simulink model "PMSM_FOC_R2026a"  (R2026a)
settings: Solver=ode4  StopTime=0.25  FixedStep=timing_h  MaxStep=1e-6
InitFcn:
  | pmsm_sensorless_v2_init(bdroot);
model workspace (MATLAB code in the model file + MAT data in the model file):
  T = 1e-6    (= 1e-06)
  MotorProfile = 'CHENSHA 200W / firmware profile revision 2'
  MotorSourceCommit = '48d6e86814ac6657b1313b4c92ef24c88f492e07'
  Pn = 200
  Un = 24
  Vdc = 24
  I_rated_rms = 11.5
  I_peak_rms = 23
  In = sqrt(2)*I_rated_rms
  I_peak = sqrt(2)*I_peak_rms
  n = 3000
  p = 5
  Rs = 0.105125
  Ld = 103.7615e-6    (= 0.0001037615)
  Lq = 103.7615e-6    (= 0.0001037615)
  Ls = Ld    (= 0.0001037615)
  phis = 0.06/(sqrt(2)*1.5*p)
  J = 32e-6    (= 3.2e-05)
  F = 0
  Kt = 1.5*p*phis
  Tn = 0.69
  T_peak = 1.38
  Iq_limit = 8
  accel_limit_rad_s2 = 1200
  speed_peak_rad_s = 335
  I_protection_A = 10
  Vbus_protection_high_V = 30
  Vbus_protection_low_V = 10
  RE = 10000
  rr = 2*pi/RE    (= 0.000628318530718)
  encoder_direction = -1
  fN = p*n/60    (= 250)
  wN = 2*pi*fN    (= 1570.79632679)
  ki_p = 0.8
  ki_i = 1
  fc = 20e3    (= 20000)
  Ts = 1/fc    (= 5e-05)
  dt = Ts    (= 5e-05)
  Ts_speed = 2*dt    (= 0.0001)
  w_sb = 2*pi*fN*1.2    (= 1884.95559215)
  fcb = 1000
  fwb = 50
  wc = 2*pi*fcb    (= 6283.18530718)
  wsc = 2*pi*fwb    (= 314.159265359)
  K = 30/pi    (= 9.54929658551)
  kp_w = 0.00069087230807625508    (= 0.000690872308076)
  ki_w = 0.04340878735241975    (= 0.0434087873524)
  ks_w = 0.98718608264211138    (= 0.987186082642)
  kp_id = 0.7539822368615503    (= 0.753982236862)
  ki_id = 879.64594300514204    (= 879.645943005)
  ks_id = 1.1309733552923253    (= 1.13097335529)
  kp_iq = 0.7539822368615503    (= 0.753982236862)
  ki_iq = 879.64594300514204    (= 879.645943005)
  ks_iq = 1.1309733552923253    (= 1.13097335529)
  Bm = 0
  uplimit_w = Kt*Iq_limit
  downlimit_w = -uplimit_w
  uplimit_id = Vdc/sqrt(3)
  downlimit_id = -uplimit_id
  uplimit_iq = Vdc/sqrt(3)
  downlimit_iq = -uplimit_iq
  teaching_Ts_speed = Ts_speed    (= 0.0001)
  teach_pwm_on = 0
  teach_pwm_cycles = 1
  decoupling_enabled = 1
  voltage_utilization = 0.96
  timing_on = 0
  timing_h = 1e-6    (= 1e-06)
  timing_control_sample = dt    (= 5e-05)
  timing_speed_sample = Ts_speed    (= 0.0001)
  timing_static_math = -1
  timing_carrier_y = [0 Ts/2 0]
  timing_adc_cfg = [0 0 0 1e-6 Ts 24.375e-6 1.1875e-6 1.5e-6 0 .5e-6 2]
  timing_pwm_cfg = [0 1e-6 Ts 24.375e-6 1.1875e-6 1.5e-6 0 5e-6 0 4000]
  dead_gate_on = 0
  dead_h = 1e-6    (= 1e-06)
  dead_gate_cfg = [0 1e-6 .5e-6]
  dead_comp_cfg = [0 .5e-6 Ts .05]
  dead_bridge_cfg = [p phis .01 0 .01 .7]
  sless_adc_mode = [1 0]
  sless_cfg = [0.105125 0.0001037615 5e-05 0.950604638176 0.469872645179 70 14 0.2 0.028048810878 0.777767679172 533.065441461 142122.303376 ... (18 elements, 1x18)]
  sless_direction = 1
  sless_enabled = 1
  sless_v2_cfg = [6.25e-08 5e-05 0.0001 2.4375e-05 1.1875e-06 1.5e-06 0 0 3e-06 5e-06 2e-06 6e-05 ... (35 elements, 1x35)]
  sless_v2_interference_s = 0
  sless_voltage_cfg = [6.25e-08 5e-05 2.8875e-05 0.105125 0.0001037615 1]
undefined symbols (not defined in the file): DiscIntNeverNeededParam
libraries: simulink x3
(part 2 of 3)

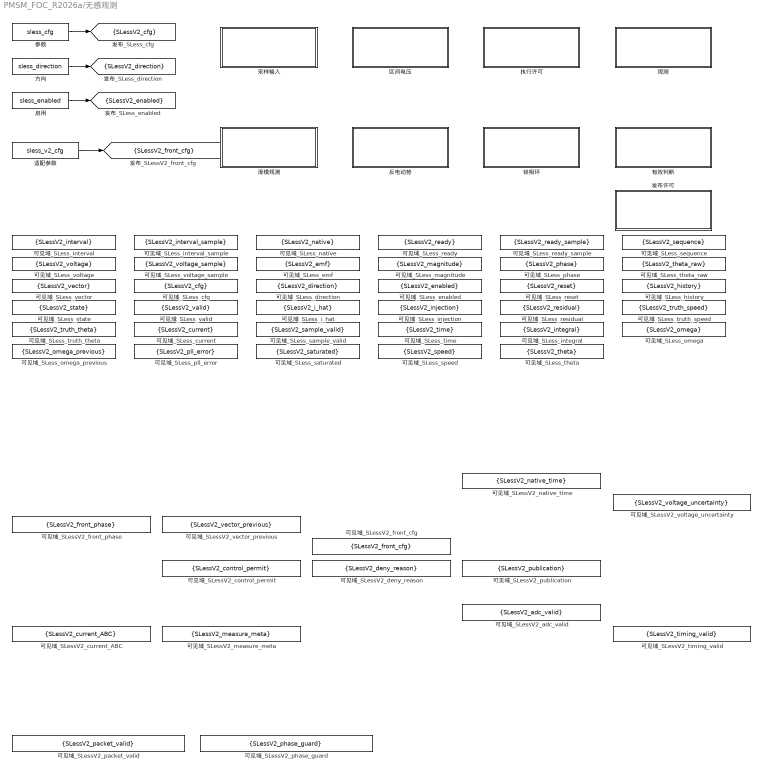
== system PMSM_FOC_R2026a/无感观测 ==
  区间电压 : Subsystem
  参数 : Constant  Value=sless_cfg  VectorParams1D=off
  反电动势 : Subsystem
  发布许可 : Subsystem
  可见域_SLessV2_adc_valid : GotoTagVisibility  GotoTag=SLessV2_adc_valid
  可见域_SLessV2_control_permit : GotoTagVisibility  GotoTag=SLessV2_control_permit
  可见域_SLessV2_current_ABC : GotoTagVisibility  GotoTag=SLessV2_current_ABC
  可见域_SLessV2_deny_reason : GotoTagVisibility  GotoTag=SLessV2_deny_reason
  可见域_SLessV2_front_cfg : GotoTagVisibility  GotoTag=SLessV2_front_cfg
  可见域_SLessV2_front_phase : GotoTagVisibility  GotoTag=SLessV2_front_phase
  可见域_SLessV2_measure_meta : GotoTagVisibility  GotoTag=SLessV2_measure_meta
  可见域_SLessV2_native_time : GotoTagVisibility  GotoTag=SLessV2_native_time
  可见域_SLessV2_packet_valid : GotoTagVisibility  GotoTag=SLessV2_packet_valid
  可见域_SLessV2_phase_guard : GotoTagVisibility  GotoTag=SLessV2_phase_guard
  可见域_SLessV2_publication : GotoTagVisibility  GotoTag=SLessV2_publication
  可见域_SLessV2_timing_valid : GotoTagVisibility  GotoTag=SLessV2_timing_valid
  可见域_SLessV2_vector_previous : GotoTagVisibility  GotoTag=SLessV2_vector_previous
  可见域_SLessV2_voltage_uncertainty : GotoTagVisibility  GotoTag=SLessV2_voltage_uncertainty
  可见域_SLess_cfg : GotoTagVisibility  GotoTag=SLessV2_cfg
  可见域_SLess_current : GotoTagVisibility  GotoTag=SLessV2_current
  可见域_SLess_direction : GotoTagVisibility  GotoTag=SLessV2_direction
  可见域_SLess_emf : GotoTagVisibility  GotoTag=SLessV2_emf
  可见域_SLess_enabled : GotoTagVisibility  GotoTag=SLessV2_enabled
  可见域_SLess_history : GotoTagVisibility  GotoTag=SLessV2_history
  可见域_SLess_i_hat : GotoTagVisibility  GotoTag=SLessV2_i_hat
  可见域_SLess_injection : GotoTagVisibility  GotoTag=SLessV2_injection
  可见域_SLess_integral : GotoTagVisibility  GotoTag=SLessV2_integral
  可见域_SLess_interval : GotoTagVisibility  GotoTag=SLessV2_interval
  可见域_SLess_interval_sample : GotoTagVisibility  GotoTag=SLessV2_interval_sample
  可见域_SLess_magnitude : GotoTagVisibility  GotoTag=SLessV2_magnitude
  可见域_SLess_native : GotoTagVisibility  GotoTag=SLessV2_native
  可见域_SLess_omega : GotoTagVisibility  GotoTag=SLessV2_omega
  可见域_SLess_omega_previous : GotoTagVisibility  GotoTag=SLessV2_omega_previous
  可见域_SLess_phase : GotoTagVisibility  GotoTag=SLessV2_phase
  可见域_SLess_pll_error : GotoTagVisibility  GotoTag=SLessV2_pll_error
  可见域_SLess_ready : GotoTagVisibility  GotoTag=SLessV2_ready
  可见域_SLess_ready_sample : GotoTagVisibility  GotoTag=SLessV2_ready_sample
  可见域_SLess_reset : GotoTagVisibility  GotoTag=SLessV2_reset
  可见域_SLess_residual : GotoTagVisibility  GotoTag=SLessV2_residual
  可见域_SLess_sample_valid : GotoTagVisibility  GotoTag=SLessV2_sample_valid
  可见域_SLess_saturated : GotoTagVisibility  GotoTag=SLessV2_saturated
  可见域_SLess_sequence : GotoTagVisibility  GotoTag=SLessV2_sequence
  可见域_SLess_speed : GotoTagVisibility  GotoTag=SLessV2_speed
  可见域_SLess_state : GotoTagVisibility  GotoTag=SLessV2_state
  可见域_SLess_theta : GotoTagVisibility  GotoTag=SLessV2_theta
  可见域_SLess_theta_raw : GotoTagVisibility  GotoTag=SLessV2_theta_raw
  可见域_SLess_time : GotoTagVisibility  GotoTag=SLessV2_time
  可见域_SLess_truth_speed : GotoTagVisibility  GotoTag=SLessV2_truth_speed
  可见域_SLess_truth_theta : GotoTagVisibility  GotoTag=SLessV2_truth_theta
  可见域_SLess_valid : GotoTagVisibility  GotoTag=SLessV2_valid
  可见域_SLess_vector : GotoTagVisibility  GotoTag=SLessV2_vector
  可见域_SLess_voltage : GotoTagVisibility  GotoTag=SLessV2_voltage
  可见域_SLess_voltage_sample : GotoTagVisibility  GotoTag=SLessV2_voltage_sample
  启用 : Constant  Value=sless_enabled  VectorParams1D=off
  执行许可 : Subsystem
  方向 : Constant  Value=sless_direction  VectorParams1D=off
  有效判断 : Subsystem
  滑模观测 : Subsystem
  观测 : Subsystem
  适配参数 : Constant  Value=sless_v2_cfg  VectorParams1D=off
  采样输入 : Subsystem
  锁相环 : Subsystem
  tag scope: SLessV2_cfg=scoped, SLessV2_direction=scoped, SLessV2_enabled=scoped, SLessV2_front_cfg=scoped
  wires:
  参数/1 -> [SLessV2_cfg]
  方向/1 -> [SLessV2_direction]
  启用/1 -> [SLessV2_enabled]
  适配参数/1 -> [SLessV2_front_cfg]

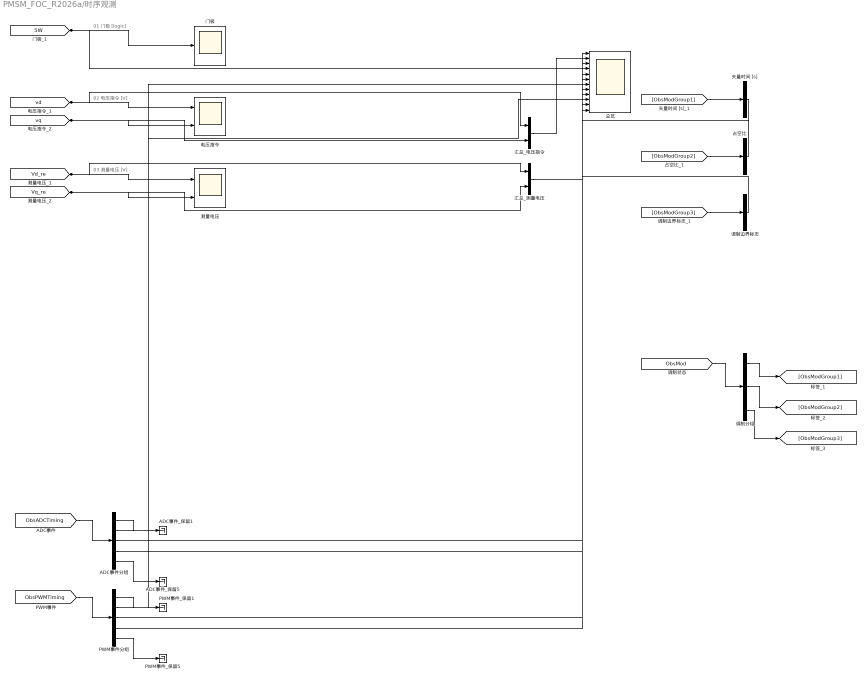
== system PMSM_FOC_R2026a/时序观测 ==
  note: 01 门极 [logic]
  note: 02 电压指令 [V]
  note: 03 测量电压 [V]
  ADC事件_保留1 : Terminator
  ADC事件_保留5 : Terminator
  ADC事件分组 : Demux  Outputs=[1 5 3 4 2]
  PWM事件_保留1 : Terminator
  PWM事件_保留5 : Terminator
  PWM事件分组 : Demux  Outputs=[2 3 3 1 3]
  占空比 : Mux  Inputs=1
  总览 : Scope  NumInputPorts=12
      settings: SampleTime=T  TimeSpan=0.12  ActiveDisplayString=12  Title=采样至生效 [s]
  汇总_测量电压 : Mux  Inputs=2
  汇总_电压指令 : Mux  Inputs=2
  测量电压 : Scope  NumInputPorts=2
      settings: SampleTime=T  Title=测量电压 [V]
  电压指令 : Scope  NumInputPorts=2
      settings: SampleTime=dt  Title=电压指令 [V]
  矢量时间 [s] : Mux  Inputs=1
  调制分组 : Demux  Outputs=[3 3 2]
  调制边界标志 : Mux  Inputs=1
  门极 : Scope
      settings: SampleTime=T  Title=门极 [logic]
  wires:
  [SW] -> 门极/1, 总览/1
  [vd] -> 电压指令/1, 汇总_电压指令/1
  [vq] -> 电压指令/2, 汇总_电压指令/2
  [Vd_re] -> 测量电压/1, 汇总_测量电压/1
  [Vq_re] -> 测量电压/2, 汇总_测量电压/2
  汇总_电压指令/1 -> 总览/2
  汇总_测量电压/1 -> 总览/3
  [ObsMod] -> 调制分组/1
  调制分组/1 -> [ObsModGroup1]
  调制分组/2 -> [ObsModGroup2]
  调制分组/3 -> [ObsModGroup3]
  [ObsModGroup1] -> 矢量时间 [s]/1
  矢量时间 [s]/1 -> 总览/4
  [ObsModGroup2] -> 占空比/1
  占空比/1 -> 总览/5
  [ObsModGroup3] -> 调制边界标志/1
  调制边界标志/1 -> 总览/6
  [ObsADCTiming] -> ADC事件分组/1
  ADC事件分组/1 -> ADC事件_保留1/1
  ADC事件分组/5 -> ADC事件_保留5/1
  [ObsPWMTiming] -> PWM事件分组/1
  PWM事件分组/1 -> PWM事件_保留1/1
  PWM事件分组/5 -> PWM事件_保留5/1
  ADC事件分组/2 -> 总览/7
  ADC事件分组/3 -> 总览/8
  ADC事件分组/4 -> 总览/9
  PWM事件分组/2 -> 总览/10
  PWM事件分组/3 -> 总览/11
  PWM事件分组/4 -> 总览/12

== system PMSM_FOC_R2026a/时序设置 ==

== system PMSM_FOC_R2026a/测量观测 ==
  note: 01 真实电流 [A]
  note: 02 测量电流 [A]
  note: 03 电角度 [rad]
  note: 04 电流误差 [A]
  note: 05 角度误差 [rad]
  总览 : Scope  NumInputPorts=5
      settings: SampleTime=dt  TimeSpan=0.12  ActiveDisplayString=5  Title=角度误差 [rad]
  汇总_电角度 : Mux  Inputs=2
  测量电流 : Scope
      settings: SampleTime=dt  Title=测量电流 [A]
  电流误差 : Scope
      settings: SampleTime=dt  Title=电流误差 [A]
  电流误差_差 : Sum  Inputs=+-
  电角度 : Scope  NumInputPorts=2
      settings: SampleTime=dt  Title=电角度 [rad]
  真实电流 : Scope
      settings: SampleTime=dt  Title=真实电流 [A]
  角度误差 : Scope
      settings: SampleTime=dt  Title=角度误差 [rad]
  角度误差_差 : Sum  Inputs=+-
  角度误差_环绕 : Fcn  Expr=atan2(sin(u(1)),cos(u(1)))
  wires:
  [Currentabc] -> 真实电流/1, 总览/1
  [Iabc_meas] -> 测量电流/1, 总览/2
  [theta_e] -> 电角度/1, 汇总_电角度/1
  [theta_meas] -> 电角度/2, 汇总_电角度/2
  [Iabc_meas] -> 电流误差_差/1
  [Currentabc] -> 电流误差_差/2
  电流误差_差/1 -> 电流误差/1, 总览/3
  [theta_meas] -> 角度误差_差/1
  [theta_e] -> 角度误差_差/2
  角度误差_差/1 -> 角度误差_环绕/1
  角度误差_环绕/1 -> 角度误差/1, 总览/5
  汇总_电角度/1 -> 总览/4

== system PMSM_FOC_R2026a/角度设置 ==
  传递延迟 : Delay  DelayLength=delay_cycles  InitialCondition=0  SampleTime=timing_control_sample
  偏置 : Constant  Value=bias_on*bias_deg*pi/180
  偏置求和 : Sum
  启用 : Constant  Value=bias_on||quant_on||delay_on
  延迟开关 : Constant  Value=delay_on
  延迟选择 : Switch  Criteria=u2 ~= 0  SaturateOnIntegerOverflow=off  InputSameDT=off
  总选择 : Switch  Criteria=u2 ~= 0  SaturateOnIntegerOverflow=off  InputSameDT=off
  最短角差 : Fcn  Expr=atan2(sin(u(1)),cos(u(1)))
  角度差 : Sum  Inputs=+-
  角度环绕 : Fcn  Expr=u(1)-2*pi*floor(u(1)/(2*pi))
  记录_log_theta_error : ToWorkspace  VariableName=log_theta_error  SaveFormat=Timeseries  SampleTime=timing_control_sample
  记录_log_theta_meas : ToWorkspace  VariableName=log_theta_meas  SaveFormat=Timeseries  SampleTime=timing_control_sample
  记录_log_theta_true : ToWorkspace  VariableName=log_theta_true  SaveFormat=Timeseries  SampleTime=timing_control_sample
  量化 : Quantizer  QuantizationInterval=step_deg*pi/180
  量化开关 : Constant  Value=quant_on
  量化选择 : Switch  Criteria=u2 ~= 0  SaturateOnIntegerOverflow=off  InputSameDT=off
  tag scope: theta_meas=global
  wires:
  [theta_e] -> 偏置求和/1, 总选择/3, 角度差/2, 记录_log_theta_true/1
  偏置/1 -> 偏置求和/2
  偏置求和/1 -> 量化/1, 量化选择/3
  量化/1 -> 量化选择/1
  量化开关/1 -> 量化选择/2
  量化选择/1 -> 角度环绕/1
  角度环绕/1 -> 传递延迟/1, 延迟选择/3
  传递延迟/1 -> 延迟选择/1
  延迟开关/1 -> 延迟选择/2
  延迟选择/1 -> 总选择/1
  启用/1 -> 总选择/2
  总选择/1 -> [theta_meas], 角度差/1, 记录_log_theta_meas/1
  角度差/1 -> 最短角差/1
  最短角差/1 -> 记录_log_theta_error/1

== system PMSM_FOC_R2026a/解耦 ==

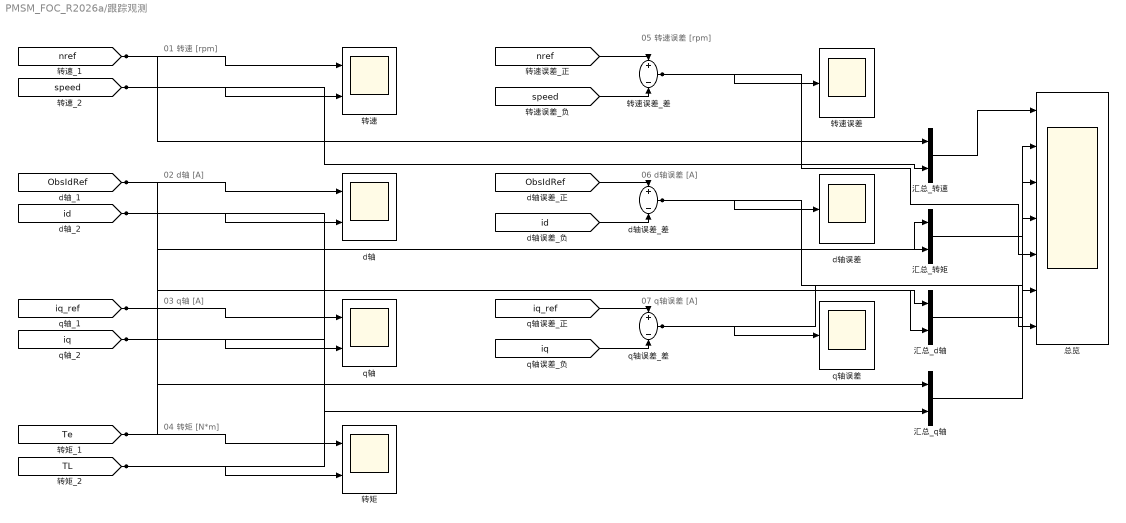
== system PMSM_FOC_R2026a/跟踪观测 ==
  note: 01 转速 [rpm]
  note: 02 d轴 [A]
  note: 03 q轴 [A]
  note: 04 转矩 [N*m]
  note: 05 转速误差 [rpm]
  note: 06 d轴误差 [A]
  note: 07 q轴误差 [A]
  d轴 : Scope  NumInputPorts=2
      settings: SampleTime=dt  Title=d轴 [A]
  d轴误差 : Scope
      settings: SampleTime=dt  Title=d轴误差 [A]
  d轴误差_差 : Sum  Inputs=+-
  q轴 : Scope  NumInputPorts=2
      settings: SampleTime=dt  Title=q轴 [A]
  q轴误差 : Scope
      settings: SampleTime=dt  Title=q轴误差 [A]
  q轴误差_差 : Sum  Inputs=+-
  总览 : Scope  NumInputPorts=7
      settings: SampleTime=dt  TimeSpan=0.12  ActiveDisplayString=7  Title=q轴误差 [A]
  汇总_d轴 : Mux  Inputs=2
  汇总_q轴 : Mux  Inputs=2
  汇总_转矩 : Mux  Inputs=2
  汇总_转速 : Mux  Inputs=2
  转矩 : Scope  NumInputPorts=2
      settings: SampleTime=dt  Title=转矩 [N*m]
  转速 : Scope  NumInputPorts=2
      settings: SampleTime=dt  Title=转速 [rpm]
  转速误差 : Scope
      settings: SampleTime=dt  Title=转速误差 [rpm]
  转速误差_差 : Sum  Inputs=+-
  wires:
  [nref] -> 转速/1, 汇总_转速/1
  [speed] -> 转速/2, 汇总_转速/2
  [ObsIdRef] -> d轴/1, 汇总_d轴/1
  [id] -> d轴/2, 汇总_d轴/2
  [iq_ref] -> q轴/1, 汇总_q轴/1
  [iq] -> q轴/2, 汇总_q轴/2
  [Te] -> 转矩/1, 汇总_转矩/1
  [TL] -> 转矩/2, 汇总_转矩/2
  [nref] -> 转速误差_差/1
  [speed] -> 转速误差_差/2
  转速误差_差/1 -> 转速误差/1, 总览/5
  [ObsIdRef] -> d轴误差_差/1
  [id] -> d轴误差_差/2
  d轴误差_差/1 -> d轴误差/1, 总览/6
  [iq_ref] -> q轴误差_差/1
  [iq] -> q轴误差_差/2
  q轴误差_差/1 -> q轴误差/1, 总览/7
  汇总_转速/1 -> 总览/1
  汇总_转矩/1 -> 总览/2
  汇总_d轴/1 -> 总览/3
  汇总_q轴/1 -> 总览/4

== system PMSM_FOC_R2026a/输出延迟 ==
  指令 : Inport
  CCR预装载 : MATLAB Function  TreatAsAtomicUnit=on
  事件时钟 : DigitalClock  SampleTime=timing_h
  启用 : Constant  Value=teach_pwm_on
  周期延迟 : Delay  DelayLength=teach_pwm_cycles  InitialCondition=0  SampleTime=timing_control_sample
  指令缓存 : UnitDelay  InitialCondition=Ts/4  SampleTime=timing_h
  时序参数 : Constant  Value=timing_pwm_cfg
  记录_log_Tcm_applied : ToWorkspace  VariableName=log_Tcm_applied  SaveFormat=Timeseries  SampleTime=timing_control_sample
  记录_log_Tcm_requested : ToWorkspace  VariableName=log_Tcm_requested  SaveFormat=Timeseries  SampleTime=timing_control_sample
  记录_obs_pwm_timing : ToWorkspace  VariableName=obs_pwm_timing  SaveFormat=Timeseries  SampleTime=timing_h
  输出方式 : VariantSource  VariantControls={real_mode==1, real_mode==0}
  选择 : Switch  Criteria=u2 ~= 0  SaturateOnIntegerOverflow=off  InputSameDT=off
  阈值向量 : Reshape
  生效 : Outport
  tag scope: ObsPWMTiming=global, SLessAppliedThreshold=global
  wires:
  指令/1 -> 周期延迟/1, 选择/3, 记录_log_Tcm_requested/1, 指令缓存/1
  周期延迟/1 -> 选择/1
  启用/1 -> 选择/2
  选择/1 -> 输出方式/2
  事件时钟/1 -> CCR预装载/1(t)
  时序参数/1 -> CCR预装载/3(cfg)
  指令缓存/1 -> CCR预装载/2(request)
  CCR预装载/1(applied) -> 阈值向量/1
  输出方式/1 -> 生效/1, 记录_log_Tcm_applied/1, [SLessAppliedThreshold]
  阈值向量/1 -> 输出方式/1
  CCR预装载/2(diag) -> 记录_obs_pwm_timing/1, [ObsPWMTiming]

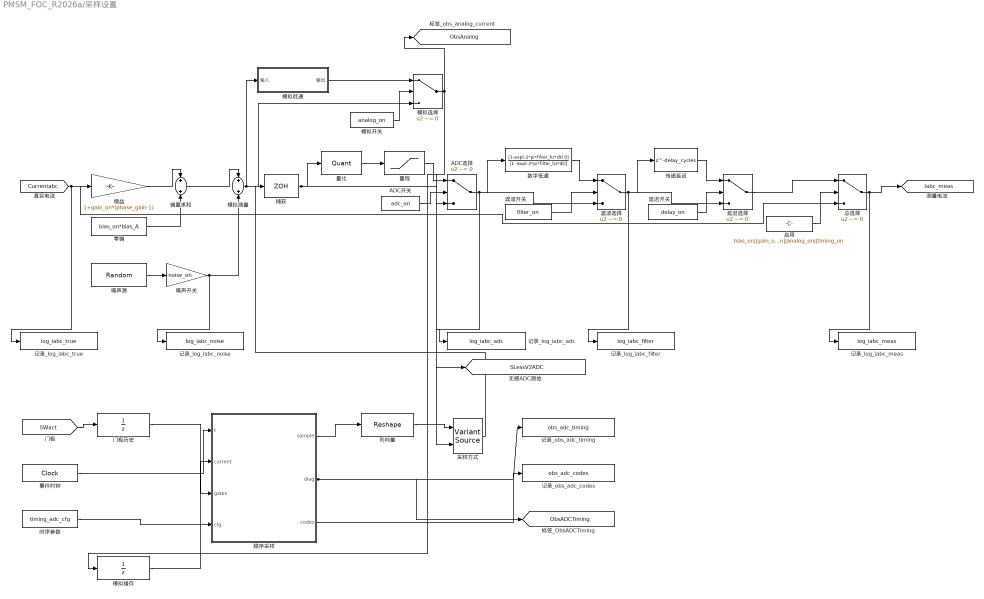
== system PMSM_FOC_R2026a/采样设置 ==
  ADC开关 : Constant  Value=adc_on
  ADC选择 : Switch  Criteria=u2 ~= 0  SaturateOnIntegerOverflow=off  InputSameDT=off
  事件时钟 : DigitalClock  SampleTime=timing_h
  传递延迟 : Delay  DelayLength=delay_cycles  InitialCondition=0  SampleTime=timing_control_sample
  偏置求和 : Sum
  列向量 : Reshape  OutputDimensionality=Column vector (2-D)
  启用 : Constant  Value=bias_on||gain_on||noise_on||adc_on||filter_on||delay_on||analog_on||timing_on
  噪声开关 : Gain  Gain=noise_on
  噪声源 : RandomNumber  Mean=[0 0 0]  Variance=noise_rms^2  Seed=noise_seed+[0 1 2]  SampleTime=timing_control_sample
  增益 : Gain  Gain=1+gain_on*(phase_gain-1)
  延迟开关 : Constant  Value=delay_on
  延迟选择 : Switch  Criteria=u2 ~= 0  SaturateOnIntegerOverflow=off  InputSameDT=off
  总选择 : Switch  Criteria=u2 ~= 0  SaturateOnIntegerOverflow=off  InputSameDT=off
  捕获 : ZeroOrderHold  SampleTime=timing_control_sample
  数字低通 : DiscreteTransferFcn  Numerator=[1-exp(-2*pi*filter_hz*dt) 0]  Denominator=[1 -exp(-2*pi*filter_hz*dt)]  SampleTime=timing_control_sample
  时序参数 : Constant  Value=timing_adc_cfg
  模拟低通 : Subsystem
  模拟开关 : Constant  Value=analog_on
  模拟测量 : Sum
  模拟缓存 : UnitDelay  InitialCondition=[0;0;0]  SampleTime=timing_h
  模拟选择 : Switch  Criteria=u2 ~= 0  SaturateOnIntegerOverflow=off  InputSameDT=off
  滤波开关 : Constant  Value=filter_on
  滤波选择 : Switch  Criteria=u2 ~= 0  SaturateOnIntegerOverflow=off  InputSameDT=off
  记录_log_iabc_adc : ToWorkspace  VariableName=log_iabc_adc  SaveFormat=Timeseries  SampleTime=timing_control_sample
  记录_log_iabc_filter : ToWorkspace  VariableName=log_iabc_filter  SaveFormat=Timeseries  SampleTime=timing_control_sample
  记录_log_iabc_meas : ToWorkspace  VariableName=log_iabc_meas  SaveFormat=Timeseries  SampleTime=timing_control_sample
  记录_log_iabc_noise : ToWorkspace  VariableName=log_iabc_noise  SaveFormat=Timeseries  SampleTime=timing_control_sample
  记录_log_iabc_true : ToWorkspace  VariableName=log_iabc_true  SaveFormat=Timeseries  SampleTime=timing_control_sample
  记录_obs_adc_codes : ToWorkspace  VariableName=obs_adc_codes  SaveFormat=Timeseries  SampleTime=timing_control_sample
  记录_obs_adc_timing : ToWorkspace  VariableName=obs_adc_timing  SaveFormat=Timeseries  SampleTime=timing_h
  采样方式 : VariantSource  VariantControls={real_mode==1, real_mode==0}
  量化 : Quantizer  QuantizationInterval=2*adc_span/2^adc_bits
  量程 : Saturate  UpperLimit=adc_span-2*adc_span/2^adc_bits  LowerLimit=-adc_span
  门极历史 : UnitDelay  InitialCondition=[0 1 0 1 0 1]  SampleTime=timing_h
  零偏 : Constant  Value=bias_on*bias_A
  顺序采样 : MATLAB Function  TreatAsAtomicUnit=on
  tag scope: Iabc_meas=global, ObsADCTiming=global, ObsAnalog=global, SLessV2ADC=global
  wires:
  [Currentabc] -> 增益/1, 总选择/3, 记录_log_iabc_true/1
  增益/1 -> 偏置求和/1
  零偏/1 -> 偏置求和/2
  偏置求和/1 -> 模拟测量/1
  噪声源/1 -> 噪声开关/1
  噪声开关/1 -> 模拟测量/2, 记录_log_iabc_noise/1
  捕获/1 -> 量化/1, ADC选择/3
  量化/1 -> 量程/1
  量程/1 -> ADC选择/1
  ADC开关/1 -> ADC选择/2
  ADC选择/1 -> 数字低通/1, 滤波选择/3, 记录_log_iabc_adc/1, [SLessV2ADC]
  数字低通/1 -> 滤波选择/1
  滤波开关/1 -> 滤波选择/2
  滤波选择/1 -> 传递延迟/1, 延迟选择/3, 记录_log_iabc_filter/1
  传递延迟/1 -> 延迟选择/1
  延迟开关/1 -> 延迟选择/2
  延迟选择/1 -> 总选择/1
  启用/1 -> 总选择/2
  总选择/1 -> [Iabc_meas], 记录_log_iabc_meas/1
  模拟测量/1 -> 模拟低通/1(输入), 模拟选择/3
  模拟低通/1(输出) -> 模拟选择/1
  模拟开关/1 -> 模拟选择/2
  模拟选择/1 -> [ObsAnalog], 模拟缓存/1, 采样方式/2
  [SWact] -> 门极历史/1
  事件时钟/1 -> 顺序采样/1(t)
  门极历史/1 -> 顺序采样/3(gates)
  时序参数/1 -> 顺序采样/4(cfg)
  模拟缓存/1 -> 顺序采样/2(current)
  顺序采样/1(sample) -> 列向量/1
  采样方式/1 -> 捕获/1
  列向量/1 -> 采样方式/1
  顺序采样/2(diag) -> 记录_obs_adc_timing/1, [ObsADCTiming]
  顺序采样/3(codes) -> 记录_obs_adc_codes/1

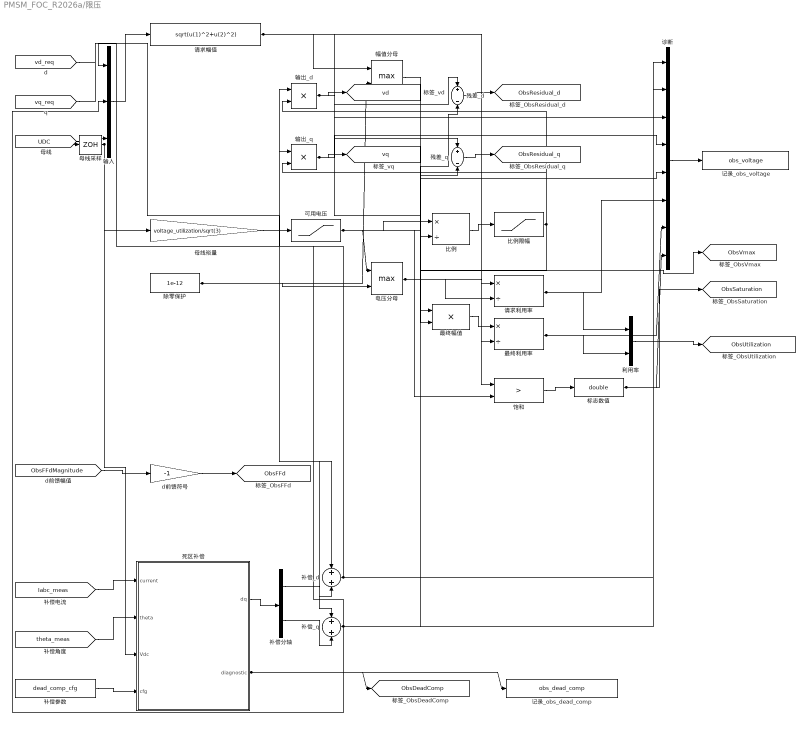
== system PMSM_FOC_R2026a/限压 ==
  d前馈符号 : Gain  Gain=-1
  利用率 : Mux  Inputs=2
  可用电压 : Saturate  UpperLimit=inf  LowerLimit=0
  幅值分母 : MinMax  Function=max  Inputs=2
  最终利用率 : Product  Inputs=*/
  最终幅值 : Product
  标志数值 : DataTypeConversion  OutDataTypeStr=double  SaturateOnIntegerOverflow=off  RndMeth=Floor
  死区补偿 : MATLAB Function  TreatAsAtomicUnit=on
  残差_d : Sum  Inputs=+-
  残差_q : Sum  Inputs=+-
  母线裕量 : Gain  Gain=voltage_utilization/sqrt(3)
  母线采样 : ZeroOrderHold  SampleTime=timing_control_sample
  比例 : Product  Inputs=*/
  比例限幅 : Saturate  UpperLimit=1  LowerLimit=0
  电压分母 : MinMax  Function=max  Inputs=2
  补偿_d : Sum
  补偿_q : Sum
  补偿分轴 : Demux  Outputs=2
  补偿参数 : Constant  Value=dead_comp_cfg
  记录_obs_dead_comp : ToWorkspace  VariableName=obs_dead_comp  SaveFormat=Timeseries  SampleTime=timing_control_sample
  记录_obs_voltage : ToWorkspace  VariableName=obs_voltage  SaveFormat=Timeseries  SampleTime=timing_control_sample
  诊断 : Mux  Inputs=8
  请求利用率 : Product  Inputs=*/
  请求幅值 : Fcn  Expr=sqrt(u(1)^2+u(2)^2)
  输入 : Mux  Inputs=3
  输出_d : Product
  输出_q : Product
  除零保护 : Constant  Value=1e-12
  饱和 : RelationalOperator  Operator=>  OutDataTypeStr=boolean  RndMeth=Simplest  InputSameDT=off
  tag scope: ObsDeadComp=global, ObsFFd=global, ObsResidual_d=global, ObsResidual_q=global, ObsSaturation=global, ObsUtilization=global, ObsVmax=global, vd=global, vq=global
  wires:
  [UDC] -> 母线采样/1
  [vd_req] -> 补偿_d/1
  [vq_req] -> 补偿_q/1
  母线采样/1 -> 输入/3, 母线裕量/1, 死区补偿/3(Vdc)
  输入/1 -> 请求幅值/1
  母线裕量/1 -> 可用电压/1
  请求幅值/1 -> 幅值分母/1, 请求利用率/1, 最终幅值/1, 饱和/1
  除零保护/1 -> 幅值分母/2, 电压分母/2
  可用电压/1 -> 电压分母/1, 比例/1, 诊断/5, 饱和/2, [ObsVmax]
  幅值分母/1 -> 比例/2
  比例/1 -> 比例限幅/1
  比例限幅/1 -> 输出_d/2, 输出_q/2, 最终幅值/2
  输出_d/1 -> [vd], 残差_d/1, 诊断/3
  残差_d/1 -> [ObsResidual_d]
  输出_q/1 -> [vq], 残差_q/1, 诊断/4
  残差_q/1 -> [ObsResidual_q]
  电压分母/1 -> 请求利用率/2, 最终利用率/2
  请求利用率/1 -> 诊断/6, 利用率/1
  最终幅值/1 -> 最终利用率/1
  最终利用率/1 -> 诊断/7, 利用率/2
  饱和/1 -> 标志数值/1
  标志数值/1 -> 诊断/8, [ObsSaturation]
  诊断/1 -> 记录_obs_voltage/1
  利用率/1 -> [ObsUtilization]
  [ObsFFdMagnitude] -> d前馈符号/1
  d前馈符号/1 -> [ObsFFd]
  [Iabc_meas] -> 死区补偿/1(current)
  [theta_meas] -> 死区补偿/2(theta)
  补偿参数/1 -> 死区补偿/4(cfg)
  死区补偿/1(dq) -> 补偿分轴/1
  补偿分轴/1 -> 补偿_d/2
  补偿_d/1 -> 输入/1, 输出_d/1, 残差_d/2, 诊断/1
  补偿分轴/2 -> 补偿_q/2
  补偿_q/1 -> 输入/2, 输出_q/1, 残差_q/2, 诊断/2
  死区补偿/2(diagnostic) -> [ObsDeadComp], 记录_obs_dead_comp/1

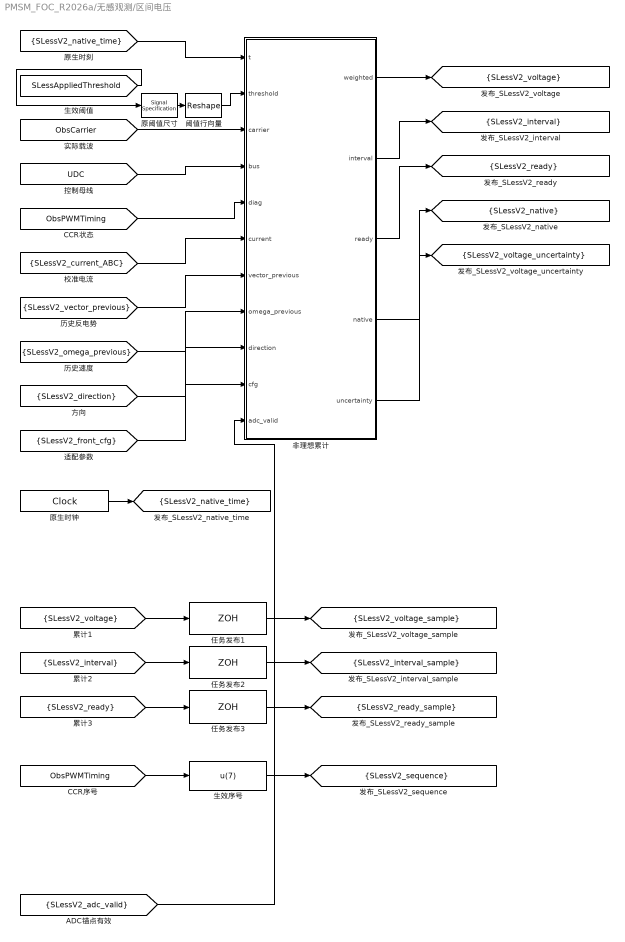
== system PMSM_FOC_R2026a/无感观测/区间电压 ==
  任务发布1 : ZeroOrderHold  SampleTime=timing_control_sample
  任务发布2 : ZeroOrderHold  SampleTime=timing_control_sample
  任务发布3 : ZeroOrderHold  SampleTime=timing_control_sample
  原生时钟 : DigitalClock  SampleTime=timing_h
  原阈值尺寸 : SignalSpecification  Dimensions=3
  生效序号 : Fcn  Expr=u(7)
  阈值行向量 : Reshape  OutputDimensionality=Row vector (2-D)
  非理想累计 : MATLAB Function  TreatAsAtomicUnit=on
  tag scope: SLessV2_interval=scoped, SLessV2_interval_sample=scoped, SLessV2_native=scoped, SLessV2_native_time=scoped, SLessV2_ready=scoped, SLessV2_ready_sample=scoped, SLessV2_sequence=scoped, SLessV2_voltage=scoped, SLessV2_voltage_sample=scoped, SLessV2_voltage_uncertainty=scoped
  wires:
  原生时钟/1 -> [SLessV2_native_time]
  [SLessV2_native_time] -> 非理想累计/1(t)
  [ObsCarrier] -> 非理想累计/3(carrier)
  [UDC] -> 非理想累计/4(bus)
  [ObsPWMTiming] -> 非理想累计/5(diag)
  [SLessV2_current_ABC] -> 非理想累计/6(current)
  [SLessV2_vector_previous] -> 非理想累计/7(vector_previous)
  [SLessV2_omega_previous] -> 非理想累计/8(omega_previous)
  [SLessV2_direction] -> 非理想累计/9(direction)
  [SLessV2_front_cfg] -> 非理想累计/10(cfg)
  [SLessAppliedThreshold] -> 原阈值尺寸/1
  原阈值尺寸/1 -> 阈值行向量/1
  阈值行向量/1 -> 非理想累计/2(threshold)
  非理想累计/1(weighted) -> [SLessV2_voltage]
  非理想累计/2(interval) -> [SLessV2_interval]
  非理想累计/3(ready) -> [SLessV2_ready]
  非理想累计/4(native) -> [SLessV2_native]
  非理想累计/5(uncertainty) -> [SLessV2_voltage_uncertainty]
  [SLessV2_voltage] -> 任务发布1/1
  任务发布1/1 -> [SLessV2_voltage_sample]
  [SLessV2_interval] -> 任务发布2/1
  任务发布2/1 -> [SLessV2_interval_sample]
  [SLessV2_ready] -> 任务发布3/1
  任务发布3/1 -> [SLessV2_ready_sample]
  [ObsPWMTiming] -> 生效序号/1
  生效序号/1 -> [SLessV2_sequence]
  [SLessV2_adc_valid] -> 非理想累计/11(adc_valid)

== system PMSM_FOC_R2026a/无感观测/反电动势 ==
  反电势历史 : UnitDelay  InitialCondition=[0;0]  SampleTime=timing_control_sample
  滤波校正 : MATLAB Function  TreatAsAtomicUnit=on
  tag scope: SLessV2_emf=scoped, SLessV2_front_phase=scoped, SLessV2_magnitude=scoped, SLessV2_phase=scoped, SLessV2_theta_raw=scoped, SLessV2_vector=scoped, SLessV2_vector_previous=scoped
  wires:
  [SLessV2_injection] -> 滤波校正/1(injection)
  [SLessV2_omega_previous] -> 滤波校正/2(omega_previous)
  [SLessV2_direction] -> 滤波校正/3(direction)
  [SLessV2_sample_valid] -> 滤波校正/4(valid)
  [SLessV2_reset] -> 滤波校正/5(reset)
  [SLessV2_cfg] -> 滤波校正/6(cfg)
  滤波校正/1(emf) -> [SLessV2_emf]
  滤波校正/2(vector) -> [SLessV2_vector]
  滤波校正/3(raw_angle) -> [SLessV2_theta_raw]
  滤波校正/4(phase) -> [SLessV2_phase]
  滤波校正/5(magnitude) -> [SLessV2_magnitude]
  [SLessV2_front_cfg] -> 滤波校正/7(front_cfg)
  滤波校正/6(front_phase) -> [SLessV2_front_phase]
  [SLessV2_vector] -> 反电势历史/1
  反电势历史/1 -> [SLessV2_vector_previous]

== system PMSM_FOC_R2026a/无感观测/发布许可 ==
  完成后发布 : MATLAB Function  TreatAsAtomicUnit=on
  tag scope: SLessV2_control_permit=scoped, SLessV2_deny_reason=scoped, SLessV2_publication=scoped
  wires:
  [SLessV2_native_time] -> 完成后发布/1(t)
  [SLessV2_theta] -> 完成后发布/2(theta)
  [SLessV2_omega] -> 完成后发布/3(omega)
  [SLessV2_packet_valid] -> 完成后发布/4(observer_valid)
  [SLessV2_adc_valid] -> 完成后发布/5(input_valid)
  [SLessV2_timing_valid] -> 完成后发布/6(timing_valid)
  [SLessV2_front_cfg] -> 完成后发布/7(cfg)
  完成后发布/1(values) -> [SLessV2_publication]
  完成后发布/2(permit) -> [SLessV2_control_permit]
  完成后发布/3(reason) -> [SLessV2_deny_reason]

== system PMSM_FOC_R2026a/无感观测/执行许可 ==
  复位 : MATLAB Function  TreatAsAtomicUnit=on
  tag scope: SLessV2_reset=scoped
  wires:
  [SLessV2_ready_sample] -> 复位/1(ready)
  [SLessV2_enabled] -> 复位/2(enabled)
  复位/1(reset) -> [SLessV2_reset]

== system PMSM_FOC_R2026a/无感观测/有效判断 ==
  瞬时相位许可 : MATLAB Function  TreatAsAtomicUnit=on
  锁定判断 : MATLAB Function  TreatAsAtomicUnit=on
  tag scope: SLessV2_history=scoped, SLessV2_packet_valid=scoped, SLessV2_phase_guard=scoped, SLessV2_state=scoped, SLessV2_valid=scoped
  wires:
  [SLessV2_residual] -> 锁定判断/1(residual)
  [SLessV2_pll_error] -> 锁定判断/2(error)
  [SLessV2_magnitude] -> 锁定判断/3(magnitude)
  [SLessV2_saturated] -> 锁定判断/4(saturated)
  [SLessV2_sample_valid] -> 锁定判断/5(sample_valid)
  [SLessV2_direction] -> 锁定判断/6(direction)
  [SLessV2_reset] -> 锁定判断/7(reset)
  [SLessV2_cfg] -> 锁定判断/8(cfg)
  锁定判断/1(valid) -> [SLessV2_valid]
  锁定判断/2(state) -> [SLessV2_state]
  锁定判断/3(history) -> [SLessV2_history]
  [SLessV2_theta] -> 瞬时相位许可/1(theta)
  [SLessV2_vector] -> 瞬时相位许可/2(vector)
  [SLessV2_valid] -> 瞬时相位许可/3(quality)
  [SLessV2_sample_valid] -> 瞬时相位许可/4(sample_valid)
  [SLessV2_reset] -> 瞬时相位许可/5(reset)
  [SLessV2_cfg] -> 瞬时相位许可/6(cfg)
  瞬时相位许可/1(packet_valid) -> [SLessV2_packet_valid]
  瞬时相位许可/2(diagnostic) -> [SLessV2_phase_guard]

== system PMSM_FOC_R2026a/无感观测/滑模观测 ==
  隐式校正 : MATLAB Function  TreatAsAtomicUnit=on
  tag scope: SLessV2_i_hat=scoped, SLessV2_injection=scoped, SLessV2_residual=scoped
  wires:
  [SLessV2_current] -> 隐式校正/1(current)
  [SLessV2_voltage_sample] -> 隐式校正/2(voltage)
  [SLessV2_sample_valid] -> 隐式校正/3(valid)
  [SLessV2_reset] -> 隐式校正/4(reset)
  [SLessV2_cfg] -> 隐式校正/5(cfg)
  隐式校正/1(estimate) -> [SLessV2_i_hat]
  隐式校正/2(residual) -> [SLessV2_residual]
  隐式校正/3(injection) -> [SLessV2_injection]

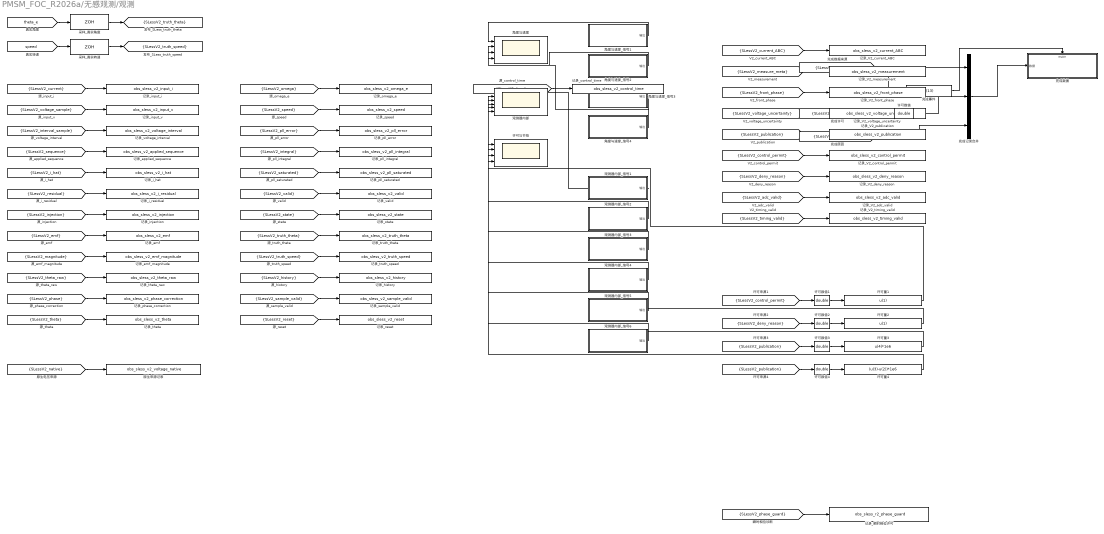
== system PMSM_FOC_R2026a/无感观测/观测 ==
  原生来源记录 : ToWorkspace  VariableName=obs_sless_v2_voltage_native  SaveFormat=Timeseries  SampleTime=timing_control_sample
  完成事件 : Fcn  Expr=u(13)
  完成数据 : Subsystem
  完成记录合并 : Mux  Inputs=3
  观测器内部 : Scope  NumInputPorts=6
      settings: OpenFcn=pmsm_sensorless_scope('open','PMSM_FOC_R2026a/无感观测/观测/观测器内部');  SampleTime=timing_control_sample  TimeSpan=0.1  TimeUnits=Metric (based on Time Span)  Title=alpha电流  YLabel=A
  观测器内部_信号1 : Subsystem
  观测器内部_信号2 : Subsystem
  观测器内部_信号3 : Subsystem
  观测器内部_信号4 : Subsystem
  观测器内部_信号5 : Subsystem
  观测器内部_信号6 : Subsystem
  角度与速度 : Scope  NumInputPorts=4
      settings: OpenFcn=pmsm_sensorless_scope('open','PMSM_FOC_R2026a/无感观测/观测/角度与速度');  SampleTime=timing_control_sample  TimeSpan=0.1  TimeUnits=Metric (based on Time Span)  Title=电角度  YLabel=°
  角度与速度_信号1 : Subsystem
  角度与速度_信号2 : Subsystem
  角度与速度_信号3 : Subsystem
  角度与速度_信号4 : Subsystem
  记录_V2_adc_valid : ToWorkspace  VariableName=obs_sless_v2_adc_valid  SaveFormat=Timeseries  SampleTime=timing_control_sample
  记录_V2_control_permit : ToWorkspace  VariableName=obs_sless_v2_control_permit  SaveFormat=Timeseries  SampleTime=timing_control_sample
  记录_V2_current_ABC : ToWorkspace  VariableName=obs_sless_v2_current_ABC  SaveFormat=Timeseries  SampleTime=timing_control_sample
  记录_V2_deny_reason : ToWorkspace  VariableName=obs_sless_v2_deny_reason  SaveFormat=Timeseries  SampleTime=timing_control_sample
  记录_V2_front_phase : ToWorkspace  VariableName=obs_sless_v2_front_phase  SaveFormat=Timeseries  SampleTime=timing_control_sample
  记录_V2_measurement : ToWorkspace  VariableName=obs_sless_v2_measurement  SaveFormat=Timeseries  SampleTime=timing_control_sample
  记录_V2_publication : ToWorkspace  VariableName=obs_sless_v2_publication  SaveFormat=Timeseries  SampleTime=timing_control_sample
  记录_V2_timing_valid : ToWorkspace  VariableName=obs_sless_v2_timing_valid  SaveFormat=Timeseries  SampleTime=timing_control_sample
  记录_V2_voltage_uncertainty : ToWorkspace  VariableName=obs_sless_v2_voltage_uncertainty  SaveFormat=Timeseries  SampleTime=timing_control_sample
  记录_applied_sequence : ToWorkspace  VariableName=obs_sless_v2_applied_sequence  SaveFormat=Timeseries  SampleTime=timing_control_sample
  记录_control_time : ToWorkspace  VariableName=obs_sless_v2_control_time  SaveFormat=Timeseries  SampleTime=timing_control_sample
  记录_emf : ToWorkspace  VariableName=obs_sless_v2_emf  SaveFormat=Timeseries  SampleTime=timing_control_sample
  记录_emf_magnitude : ToWorkspace  VariableName=obs_sless_v2_emf_magnitude  SaveFormat=Timeseries  SampleTime=timing_control_sample
  记录_history : ToWorkspace  VariableName=obs_sless_v2_history  SaveFormat=Timeseries  SampleTime=timing_control_sample
  记录_i_hat : ToWorkspace  VariableName=obs_sless_v2_i_hat  SaveFormat=Timeseries  SampleTime=timing_control_sample
  记录_i_residual : ToWorkspace  VariableName=obs_sless_v2_i_residual  SaveFormat=Timeseries  SampleTime=timing_control_sample
  记录_injection : ToWorkspace  VariableName=obs_sless_v2_injection  SaveFormat=Timeseries  SampleTime=timing_control_sample
  记录_input_i : ToWorkspace  VariableName=obs_sless_v2_input_i  SaveFormat=Timeseries  SampleTime=timing_control_sample
  记录_input_v : ToWorkspace  VariableName=obs_sless_v2_input_v  SaveFormat=Timeseries  SampleTime=timing_control_sample
  记录_omega_e : ToWorkspace  VariableName=obs_sless_v2_omega_e  SaveFormat=Timeseries  SampleTime=timing_control_sample
  记录_phase_correction : ToWorkspace  VariableName=obs_sless_v2_phase_correction  SaveFormat=Timeseries  SampleTime=timing_control_sample
  记录_pll_error : ToWorkspace  VariableName=obs_sless_v2_pll_error  SaveFormat=Timeseries  SampleTime=timing_control_sample
  记录_pll_integral : ToWorkspace  VariableName=obs_sless_v2_pll_integral  SaveFormat=Timeseries  SampleTime=timing_control_sample
  记录_pll_saturated : ToWorkspace  VariableName=obs_sless_v2_pll_saturated  SaveFormat=Timeseries  SampleTime=timing_control_sample
  记录_reset : ToWorkspace  VariableName=obs_sless_v2_reset  SaveFormat=Timeseries  SampleTime=timing_control_sample
  记录_sample_valid : ToWorkspace  VariableName=obs_sless_v2_sample_valid  SaveFormat=Timeseries  SampleTime=timing_control_sample
  记录_speed : ToWorkspace  VariableName=obs_sless_v2_speed  SaveFormat=Timeseries  SampleTime=timing_control_sample
  记录_state : ToWorkspace  VariableName=obs_sless_v2_state  SaveFormat=Timeseries  SampleTime=timing_control_sample
  记录_theta : ToWorkspace  VariableName=obs_sless_v2_theta  SaveFormat=Timeseries  SampleTime=timing_control_sample
  记录_theta_raw : ToWorkspace  VariableName=obs_sless_v2_theta_raw  SaveFormat=Timeseries  SampleTime=timing_control_sample
  记录_truth_speed : ToWorkspace  VariableName=obs_sless_v2_truth_speed  SaveFormat=Timeseries  SampleTime=timing_control_sample
  记录_truth_theta : ToWorkspace  VariableName=obs_sless_v2_truth_theta  SaveFormat=Timeseries  SampleTime=timing_control_sample
  记录_valid : ToWorkspace  VariableName=obs_sless_v2_valid  SaveFormat=Timeseries  SampleTime=timing_control_sample
  记录_voltage_interval : ToWorkspace  VariableName=obs_sless_v2_voltage_interval  SaveFormat=Timeseries  SampleTime=timing_control_sample
  记录_瞬时相位许可 : ToWorkspace  VariableName=obs_sless_r2_phase_guard  SaveFormat=Timeseries  SampleTime=timing_control_sample
  许可与节拍 : Scope  NumInputPorts=4
      settings: SampleTime=timing_control_sample  TimeSpan=0.005  Title=控制许可
  许可数值{,1..4} (5 alike) : DataTypeConversion  OutDataTypeStr=double  SaturateOnIntegerOverflow=off  RndMeth=Floor
  许可量1 : Fcn  Expr=u(1)
  许可量2 : Fcn  Expr=u(1)
  许可量3 : Fcn  Expr=u(4)*1e6
  许可量4 : Fcn  Expr=(u(3)-u(2))*1e6
  采样_真实角度 : ZeroOrderHold  SampleTime=timing_control_sample
  采样_真实转速 : ZeroOrderHold  SampleTime=timing_control_sample
  tag scope: SLessV2_truth_speed=scoped, SLessV2_truth_theta=scoped
  wires:
  [theta_e] -> 采样_真实角度/1
  采样_真实角度/1 -> [SLessV2_truth_theta]
  [speed] -> 采样_真实转速/1
  采样_真实转速/1 -> [SLessV2_truth_speed]
  [SLessV2_current] -> 记录_input_i/1
  [SLessV2_voltage_sample] -> 记录_input_v/1
  [SLessV2_interval_sample] -> 记录_voltage_interval/1
  [SLessV2_sequence] -> 记录_applied_sequence/1
  [SLessV2_i_hat] -> 记录_i_hat/1
  [SLessV2_residual] -> 记录_i_residual/1
  [SLessV2_injection] -> 记录_injection/1
  [SLessV2_emf] -> 记录_emf/1
  [SLessV2_magnitude] -> 记录_emf_magnitude/1
  [SLessV2_theta_raw] -> 记录_theta_raw/1
  [SLessV2_phase] -> 记录_phase_correction/1
  [SLessV2_theta] -> 记录_theta/1
  [SLessV2_omega] -> 记录_omega_e/1
  [SLessV2_speed] -> 记录_speed/1
  [SLessV2_pll_error] -> 记录_pll_error/1
  [SLessV2_integral] -> 记录_pll_integral/1
  [SLessV2_saturated] -> 记录_pll_saturated/1
  [SLessV2_valid] -> 记录_valid/1
  [SLessV2_state] -> 记录_state/1
  [SLessV2_truth_theta] -> 记录_truth_theta/1
  [SLessV2_truth_speed] -> 记录_truth_speed/1
  [SLessV2_history] -> 记录_history/1
  [SLessV2_sample_valid] -> 记录_sample_valid/1
  [SLessV2_reset] -> 记录_reset/1
  [SLessV2_time] -> 记录_control_time/1
  [SLessV2_native] -> 原生来源记录/1
  角度与速度_信号1/1(输出) -> 角度与速度/1
  角度与速度_信号2/1(输出) -> 角度与速度/2
  角度与速度_信号3/1(输出) -> 角度与速度/3
  角度与速度_信号4/1(输出) -> 角度与速度/4
  观测器内部_信号1/1(输出) -> 观测器内部/1
  观测器内部_信号2/1(输出) -> 观测器内部/2
  观测器内部_信号3/1(输出) -> 观测器内部/3
  观测器内部_信号4/1(输出) -> 观测器内部/4
  观测器内部_信号5/1(输出) -> 观测器内部/5
  观测器内部_信号6/1(输出) -> 观测器内部/6
  [SLessV2_current_ABC] -> 记录_V2_current_ABC/1
  [SLessV2_measure_meta] -> 记录_V2_measurement/1
  [SLessV2_front_phase] -> 记录_V2_front_phase/1
  [SLessV2_voltage_uncertainty] -> 记录_V2_voltage_uncertainty/1
  [SLessV2_publication] -> 记录_V2_publication/1
  [SLessV2_control_permit] -> 记录_V2_control_permit/1
  [SLessV2_deny_reason] -> 记录_V2_deny_reason/1
  [SLessV2_adc_valid] -> 记录_V2_adc_valid/1
  [SLessV2_timing_valid] -> 记录_V2_timing_valid/1
  [SLessV2_control_permit] -> 许可数值1/1
  许可数值1/1 -> 许可量1/1
  许可量1/1 -> 许可与节拍/1
  [SLessV2_deny_reason] -> 许可数值2/1
  许可数值2/1 -> 许可量2/1
  许可量2/1 -> 许可与节拍/2
  [SLessV2_publication] -> 许可数值3/1
  许可数值3/1 -> 许可量3/1
  许可量3/1 -> 许可与节拍/3
  [SLessV2_publication] -> 许可数值4/1
  许可数值4/1 -> 许可量4/1
  许可量4/1 -> 许可与节拍/4
  [SLessV2_phase_guard] -> 记录_瞬时相位许可/1
  [SLessV2_publication] -> 完成记录合并/1, 完成事件/1
  [SLessV2_control_permit] -> 许可数值/1
  许可数值/1 -> 完成记录合并/2
  [SLessV2_deny_reason] -> 完成记录合并/3
  完成记录合并/1 -> 完成数据/1(数据)
  完成事件/1 -> 完成数据/Enable

== system PMSM_FOC_R2026a/无感观测/采样输入 ==
  任务时钟 : DigitalClock  SampleTime=timing_control_sample
  原始ADC_列向量 : Reshape  OutputDimensionality=Column vector (2-D)
  原始ADC_原尺寸 : SignalSpecification  Dimensions=[3 1]
  校准对齐 : MATLAB Function  TreatAsAtomicUnit=on
  滤后测量_列向量 : Reshape  OutputDimensionality=Column vector (2-D)
  滤后测量_原尺寸 : SignalSpecification  Dimensions=[3 1]
  tag scope: SLessV2_adc_valid=scoped, SLessV2_current=scoped, SLessV2_current_ABC=scoped, SLessV2_measure_meta=scoped, SLessV2_sample_valid=scoped, SLessV2_time=scoped, SLessV2_timing_valid=scoped
  wires:
  任务时钟/1 -> [SLessV2_time]
  [SLessV2_time] -> 校准对齐/1(t)
  [ObsADCTiming] -> 校准对齐/4(diag)
  [SLessV2_front_cfg] -> 校准对齐/5(cfg)
  [Iabc_meas] -> 滤后测量_原尺寸/1
  滤后测量_原尺寸/1 -> 滤后测量_列向量/1
  滤后测量_列向量/1 -> 校准对齐/2(measured)
  [SLessV2ADC] -> 原始ADC_原尺寸/1
  原始ADC_原尺寸/1 -> 原始ADC_列向量/1
  原始ADC_列向量/1 -> 校准对齐/3(adc)
  校准对齐/1(current) -> [SLessV2_current]
  校准对齐/2(calibrated) -> [SLessV2_current_ABC]
  校准对齐/3(valid) -> [SLessV2_sample_valid]
  校准对齐/4(adc_valid) -> [SLessV2_adc_valid]
  校准对齐/5(timing_valid) -> [SLessV2_timing_valid]
  校准对齐/6(meta) -> [SLessV2_measure_meta]

== system PMSM_FOC_R2026a/无感观测/锁相环 ==
  归一化PLL : MATLAB Function  TreatAsAtomicUnit=on
  速度历史 : UnitDelay  SampleTime=timing_control_sample
  tag scope: SLessV2_integral=scoped, SLessV2_omega=scoped, SLessV2_omega_previous=scoped, SLessV2_pll_error=scoped, SLessV2_saturated=scoped, SLessV2_speed=scoped, SLessV2_theta=scoped
  wires:
  [SLessV2_vector] -> 归一化PLL/1(vector)
  [SLessV2_magnitude] -> 归一化PLL/2(magnitude)
  [SLessV2_direction] -> 归一化PLL/3(direction)
  [SLessV2_sample_valid] -> 归一化PLL/4(valid)
  [SLessV2_reset] -> 归一化PLL/5(reset)
  [SLessV2_enabled] -> 归一化PLL/6(enabled)
  [SLessV2_cfg] -> 归一化PLL/7(cfg)
  归一化PLL/1(theta) -> [SLessV2_theta]
  归一化PLL/2(omega) -> [SLessV2_omega]
  归一化PLL/3(error) -> [SLessV2_pll_error]
  归一化PLL/4(integral) -> [SLessV2_integral]
  归一化PLL/5(saturated) -> [SLessV2_saturated]
  归一化PLL/6(speed) -> [SLessV2_speed]
  [SLessV2_omega] -> 速度历史/1
  速度历史/1 -> [SLessV2_omega_previous]

== system PMSM_FOC_R2026a/采样设置/模拟低通 ==
  输入 : Inport
  RC1 : TransferFcn  Numerator=[2*pi*analog_hz]  Denominator=[1 2*pi*analog_hz]
  RC2 : TransferFcn  Numerator=[2*pi*analog_hz]  Denominator=[1 2*pi*analog_hz]
  RC3 : TransferFcn  Numerator=[2*pi*analog_hz]  Denominator=[1 2*pi*analog_hz]
  分相 : Demux  Outputs=3
  合相 : Mux  Inputs=3
  输出 : Outport
  wires:
  输入/1 -> 分相/1
  合相/1 -> 输出/1
  分相/1 -> RC1/1
  RC1/1 -> 合相/1
  分相/2 -> RC2/1
  RC2/1 -> 合相/2
  分相/3 -> RC3/1
  RC3/1 -> 合相/3

== system PMSM_FOC_R2026a/无感观测/观测/完成数据 ==
  数据 : Inport  PortDimensions=[15 1]
  完成 : EnablePort
  保存 : ToWorkspace  VariableName=obs_sless_direct_completed  SaveFormat=Timeseries  SampleTime=-1
  wires:
  数据/1 -> 保存/1

== system PMSM_FOC_R2026a/无感观测/观测/观测器内部_信号1 ==
  合并 : BusCreator  Inputs=2
  数值1 : DataTypeConversion  OutDataTypeStr=double  SaturateOnIntegerOverflow=off  RndMeth=Floor
  数值2 : DataTypeConversion  OutDataTypeStr=double  SaturateOnIntegerOverflow=off  RndMeth=Floor
  通道1 : Fcn  Expr=u(1)*1
  通道2 : Fcn  Expr=u(1)*1
  输出 : Outport
  wires:
  [SLessV2_current] -> 数值1/1
  数值1/1 -> 通道1/1
  通道1/1 -> 合并/1  "测量"
  [SLessV2_i_hat] -> 数值2/1
  数值2/1 -> 通道2/1
  通道2/1 -> 合并/2  "估计"
  合并/1 -> 输出/1

== system PMSM_FOC_R2026a/无感观测/观测/观测器内部_信号2 ==
  合并 : BusCreator  Inputs=2
  数值1 : DataTypeConversion  OutDataTypeStr=double  SaturateOnIntegerOverflow=off  RndMeth=Floor
  数值2 : DataTypeConversion  OutDataTypeStr=double  SaturateOnIntegerOverflow=off  RndMeth=Floor
  通道1 : Fcn  Expr=u(2)*1
  通道2 : Fcn  Expr=u(2)*1
  输出 : Outport
  wires:
  [SLessV2_current] -> 数值1/1
  数值1/1 -> 通道1/1
  通道1/1 -> 合并/1  "测量"
  [SLessV2_i_hat] -> 数值2/1
  数值2/1 -> 通道2/1
  通道2/1 -> 合并/2  "估计"
  合并/1 -> 输出/1

== system PMSM_FOC_R2026a/无感观测/观测/观测器内部_信号3 ==
  合并 : BusCreator  Inputs=2
  数值1 : DataTypeConversion  OutDataTypeStr=double  SaturateOnIntegerOverflow=off  RndMeth=Floor
  数值2 : DataTypeConversion  OutDataTypeStr=double  SaturateOnIntegerOverflow=off  RndMeth=Floor
  通道1 : Fcn  Expr=u(1)*1
  通道2 : Fcn  Expr=u(2)*1
  输出 : Outport
  wires:
  [SLessV2_emf] -> 数值1/1
  数值1/1 -> 通道1/1
  通道1/1 -> 合并/1  "alpha"
  [SLessV2_emf] -> 数值2/1
  数值2/1 -> 通道2/1
  通道2/1 -> 合并/2  "beta"
  合并/1 -> 输出/1

== system PMSM_FOC_R2026a/无感观测/观测/观测器内部_信号4 ==
  合并 : BusCreator  Inputs=1
  数值1 : DataTypeConversion  OutDataTypeStr=double  SaturateOnIntegerOverflow=off  RndMeth=Floor
  通道1 : Fcn  Expr=u(1)*1
  输出 : Outport
  wires:
  [SLessV2_pll_error] -> 数值1/1
  数值1/1 -> 通道1/1
  通道1/1 -> 合并/1  "鉴相误差"
  合并/1 -> 输出/1

== system PMSM_FOC_R2026a/无感观测/观测/观测器内部_信号5 ==
  合并 : BusCreator  Inputs=1
  数值1 : DataTypeConversion  OutDataTypeStr=double  SaturateOnIntegerOverflow=off  RndMeth=Floor
  通道1 : Fcn  Expr=u(1)*1
  输出 : Outport
  wires:
  [SLessV2_integral] -> 数值1/1
  数值1/1 -> 通道1/1
  通道1/1 -> 合并/1  "积分"
  合并/1 -> 输出/1

== system PMSM_FOC_R2026a/无感观测/观测/观测器内部_信号6 ==
  合并 : BusCreator  Inputs=1
  数值1 : DataTypeConversion  OutDataTypeStr=double  SaturateOnIntegerOverflow=off  RndMeth=Floor
  通道1 : Fcn  Expr=u(1)*57.295779513082323
  输出 : Outport
  wires:
  [SLessV2_phase] -> 数值1/1
  数值1/1 -> 通道1/1
  通道1/1 -> 合并/1  "校正"
  合并/1 -> 输出/1

== system PMSM_FOC_R2026a/无感观测/观测/角度与速度_信号1 ==
  合并 : BusCreator  Inputs=2
  数值1 : DataTypeConversion  OutDataTypeStr=double  SaturateOnIntegerOverflow=off  RndMeth=Floor
  数值2 : DataTypeConversion  OutDataTypeStr=double  SaturateOnIntegerOverflow=off  RndMeth=Floor
  通道1 : Fcn  Expr=u(1)*57.295779513082323
  通道2 : Fcn  Expr=u(1)*57.295779513082323
  输出 : Outport
  wires:
  [SLessV2_truth_theta] -> 数值1/1
  数值1/1 -> 通道1/1
  通道1/1 -> 合并/1  "真值"
  [SLessV2_theta] -> 数值2/1
  数值2/1 -> 通道2/1
  通道2/1 -> 合并/2  "估计"
  合并/1 -> 输出/1

== system PMSM_FOC_R2026a/无感观测/观测/角度与速度_信号2 ==
  合并 : BusCreator  Inputs=2
  数值1 : DataTypeConversion  OutDataTypeStr=double  SaturateOnIntegerOverflow=off  RndMeth=Floor
  数值2 : DataTypeConversion  OutDataTypeStr=double  SaturateOnIntegerOverflow=off  RndMeth=Floor
  通道1 : Fcn  Expr=u(1)*1
  通道2 : Fcn  Expr=u(1)*1
  输出 : Outport
  wires:
  [SLessV2_truth_speed] -> 数值1/1
  数值1/1 -> 通道1/1
  通道1/1 -> 合并/1  "真值"
  [SLessV2_speed] -> 数值2/1
  数值2/1 -> 通道2/1
  通道2/1 -> 合并/2  "估计"
  合并/1 -> 输出/1

== system PMSM_FOC_R2026a/无感观测/观测/角度与速度_信号3 ==
  合并 : Mux  Inputs=2
  数值1 : DataTypeConversion  OutDataTypeStr=double  SaturateOnIntegerOverflow=off  RndMeth=Floor
  数值2 : DataTypeConversion  OutDataTypeStr=double  SaturateOnIntegerOverflow=off  RndMeth=Floor
  环绕误差 : Fcn  Expr=atan2(sin(u(1)-u(2)),cos(u(1)-u(2)))*180/pi
  通道1 : Fcn  Expr=u(1)
  通道2 : Fcn  Expr=u(1)
  输出 : Outport
  wires:
  [SLessV2_theta] -> 数值1/1
  数值1/1 -> 通道1/1
  通道1/1 -> 合并/1  "估计"
  [SLessV2_truth_theta] -> 数值2/1
  数值2/1 -> 通道2/1
  通道2/1 -> 合并/2  "真值"
  合并/1 -> 环绕误差/1
  环绕误差/1 -> 输出/1

== system PMSM_FOC_R2026a/无感观测/观测/角度与速度_信号4 ==
  合并 : BusCreator  Inputs=3
  数值1 : DataTypeConversion  OutDataTypeStr=double  SaturateOnIntegerOverflow=off  RndMeth=Floor
  数值2 : DataTypeConversion  OutDataTypeStr=double  SaturateOnIntegerOverflow=off  RndMeth=Floor
  数值3 : DataTypeConversion  OutDataTypeStr=double  SaturateOnIntegerOverflow=off  RndMeth=Floor
  通道1 : Fcn  Expr=u(1)*1
  通道2 : Fcn  Expr=u(1)*1
  通道3 : Fcn  Expr=u(1)*1
  输出 : Outport
  wires:
  [SLessV2_valid] -> 数值1/1
  数值1/1 -> 通道1/1
  通道1/1 -> 合并/1  "观测锁定"
  [SLessV2_state] -> 数值2/1
  数值2/1 -> 通道2/1
  通道2/1 -> 合并/2  "状态"
  [SLessV2_saturated] -> 数值3/1
  数值3/1 -> 通道3/1
  通道3/1 -> 合并/3  "饱和"
  合并/1 -> 输出/1

== matlab function PMSM_FOC_R2026a/无感观测/区间电压/非理想累计 ==
  settings: updateMethod=DISCRETE  sampleTime=timing_h
  data: t input double size=1; weighted output double size=[2 1]; threshold input double size=[1 3]; carrier input double size=1; bus input double size=1; diag input double size=[1 12]; current input double size=[3 1]; vector_previous input double size=[2 1]; omega_previous input double size=1; direction input double size=1; cfg input double size=[1 35]; interval output double size=[2 1]; ready output boolean size=1; native output double size=[36 1]; uncertainty output double size=[2 1]; adc_valid input boolean size=1
function [weighted,interval,ready,native,uncertainty]=sless_direct_voltage_block(t,threshold,carrier,bus,diag,current,vector_previous,omega_previous,direction,cfg,adc_valid)
%#codegen
% Reuse the causal voltage equations; only valid ADC data can anchor them.
persistent s
if isempty(s),s=sensorless_v2_voltage_state;end
c=sensorless_v2_config_rt(cfg);
[s,weighted,interval,ready,native,uncertainty]=sensorless_r2_voltage_step(s,t,threshold,carrier,bus,diag(7),current,vector_previous,omega_previous,direction,c,adc_valid);
end

== matlab function PMSM_FOC_R2026a/无感观测/执行许可/复位 ==
  settings: updateMethod=DISCRETE  sampleTime=timing_control_sample
  data: ready input boolean size=1; reset output boolean size=1; enabled input double size=1
function reset=sless_reset_block(ready,enabled)
%#codegen
reset=~ready||enabled==0;
end

== matlab function PMSM_FOC_R2026a/无感观测/滑模观测/隐式校正 ==
  settings: updateMethod=DISCRETE  sampleTime=timing_control_sample
  data: current input double size=[2 1]; estimate output double size=[2 1]; voltage input double size=[2 1]; valid input boolean size=1; reset input boolean size=1; cfg input double size=[1 18]; residual output double size=[2 1]; injection output double size=[2 1]
function [estimate,residual,injection]=sless_smo_block(current,voltage,valid,reset,cfg)
%#codegen
persistent previous
if isempty(previous),previous=struct('i',zeros(2,1),'z',zeros(2,1));end
c=sensorless_rt_config(cfg);
[previous,diag]=sensorless_smo_step(previous,current,voltage,c,valid,reset);
estimate=previous.i;residual=diag.residual;injection=previous.z;
end

== matlab function PMSM_FOC_R2026a/无感观测/反电动势/滤波校正 ==
  settings: updateMethod=DISCRETE  sampleTime=timing_control_sample
  data: injection input double size=[2 1]; emf output double size=[2 1]; omega_previous input double size=1; direction input double size=1; valid input boolean size=1; reset input boolean size=1; cfg input double size=[1 18]; vector output double size=[2 1]; raw_angle output double size=1; phase output double size=1; magnitude output double size=1; front_cfg input double size=[1 35]; front_phase output double size=1
function [emf,vector,raw_angle,phase,magnitude,front_phase]=sless_v2_emf_block(injection,omega_previous,direction,valid,reset,cfg,front_cfg)
%#codegen
persistent previous
if isempty(previous),previous=zeros(2,1);end
c=sensorless_rt_config(cfg);f=sensorless_v2_config_rt(front_cfg);
if reset,omega_previous=0;end
[previous,d]=sensorless_emf_step(previous,injection,omega_previous,direction,c,valid,reset);
[front_phase,~]=sensorless_v2_front_phase(omega_previous,f);
emf=previous;rotation=[cos(front_phase) -sin(front_phase);sin(front_phase) cos(front_phase)];
vector=rotation*d.vector;raw_angle=d.raw_theta;phase=d.phase_correction;magnitude=d.magnitude;
end

== matlab function PMSM_FOC_R2026a/无感观测/锁相环/归一化PLL ==
  settings: updateMethod=DISCRETE  sampleTime=timing_control_sample
  data: vector input double size=[2 1]; theta output double size=1; magnitude input double size=1; direction input double size=1; valid input boolean size=1; reset input boolean size=1; enabled input double size=1; cfg input double size=[1 18]; omega output double size=1; error output double size=1; integral output double size=1; saturated output boolean size=1; speed output double size=1
function [theta,omega,error,integral,saturated,speed]=sless_pll_block(vector,magnitude,direction,valid,reset,enabled,cfg)
%#codegen
persistent previous
if isempty(previous),previous=struct('theta',0,'integral',0,'omega',0);end
c=sensorless_rt_config(cfg);
permission=enabled~=0&&valid&&direction~=0&&magnitude>=c.validity.emf_off_below_V;
[previous,diag]=sensorless_pll_step(previous,vector,c,permission,reset);
theta=diag.theta;omega=diag.omega;error=diag.error;
integral=diag.integral;saturated=diag.saturated;speed=omega/c.pole_pairs*60/(2*pi);
end

== matlab function PMSM_FOC_R2026a/无感观测/有效判断/锁定判断 ==
  settings: updateMethod=DISCRETE  sampleTime=timing_control_sample
  data: residual input double size=[2 1]; valid output boolean size=1; error input double size=1; magnitude input double size=1; saturated input boolean size=1; sample_valid input boolean size=1; direction input double size=1; reset input boolean size=1; cfg input double size=[1 18]; state output double size=1; history output double size=[3 1]
function [valid,state,history]=sless_validity_block(residual,error,magnitude,saturated,sample_valid,direction,reset,cfg)
%#codegen
persistent previous
c=sensorless_rt_config(cfg);
if isempty(previous),previous=sensorless_state(c);end
[previous,valid,state]=sensorless_validity_step(previous,residual,error,magnitude,saturated,sample_valid,direction,reset,c);
history=[previous.lock_count;previous.history_count;previous.unlock_count];
end

== matlab function PMSM_FOC_R2026a/无感观测/发布许可/完成后发布 ==
  settings: updateMethod=DISCRETE  sampleTime=timing_h
  data: t input double size=1; values output double size=[13 1]; theta input double size=1; omega input double size=1; observer_valid input boolean size=1; input_valid input boolean size=1; timing_valid input boolean size=1; cfg input double size=[1 35]; permit output boolean size=1; reason output double size=1
function [values,permit,reason]=sless_direct_queue_block(t,theta,omega,observer_valid,input_valid,timing_valid,cfg)
%#codegen
% Normal JEOS capture and delayed publication, without injected events.
persistent queue integrity_latched
if isempty(queue),queue=sensorless_v2_queue_state;integrity_latched=false;end
c=sensorless_v2_config_rt(cfg);tick=round(t/c.h_s);N=round(c.period_s/c.h_s);
first=round((c.adc_trigger_s+c.adc_sync_s+3*c.adc_rank_s)/c.h_s);
new_capture=tick>=first&&mod(tick-first,N)==0&&tick~=queue.last_capture;
[queue,values,permit,reason]=sensorless_v2_queue_step(queue,t,theta,omega,observer_valid,input_valid,timing_valid,c);
if new_capture&&queue.has_pending
 queue.pending.available_time_s=(tick+ceil(c.observer_exec_s/c.h_s-1e-9))*c.h_s;
end
if bitand(uint16(reason),uint16(96))~=0,integrity_latched=true;end
if integrity_latched,permit=false;reason=double(bitor(uint16(reason),uint16(4096)));end
if ~permit,values(9:11)=0;end
end

== matlab function PMSM_FOC_R2026a/采样设置/顺序采样 ==
  settings: updateMethod=DISCRETE  sampleTime=timing_h
  data: t input; sample output size=[1 3]; current input; gates input; cfg input; diag output size=[1 15]; codes output size=[1 3]
function [sample,diag,codes] = timing_adc(t,current,gates,cfg)
%#codegen
% cfg: on, window, hold-invalid, h, Ts, trigger, aperture, rank, sync, guard, speed divider.
% Quantized event grid; outputs are published together at JEOS, in A/B/C order.
persistent captured delivered valid elapsed aperture_ok last_good raw_codes
if isempty(captured)
 captured=zeros(1,3);delivered=zeros(1,3);valid=zeros(1,3);
 elapsed=zeros(1,3);aperture_ok=ones(1,3);last_good=zeros(1,3);raw_codes=2048*ones(1,3);
end
sample=delivered;codes=raw_codes;diag=zeros(1,15);
if cfg(1)==0,return;end
h=cfg(4);N=round(cfg(5)/h);tick=round(t/h);phase=mod(tick,N);
tr=round((cfg(6)+cfg(9))/h);ap=round(cfg(7)/h);rank=round(cfg(8)/h);
guard=ceil(cfg(10)/h);pulse=zeros(1,5);
if phase==tr,pulse(1)=1;end
for k=1:3
 % Gates are sampled one grid tick earlier to avoid an algebraic gate loop.
 if gates(2*k)>0.5,elapsed(k)=elapsed(k)+1;else,elapsed(k)=0;end
 r=3-k;start=tr+r*rank;finish=start+ap;
 if phase==start,aperture_ok(k)=double(elapsed(k)>guard);end
 if phase>=start && phase<=finish && elapsed(k)<=guard,aperture_ok(k)=0;end
 if phase==finish
  valid(k)=aperture_ok(k);pulse(r+2)=1;
 end
 % Input read buffer is one tick old. Read on the following tick so the
 % captured physical value remains exactly at the aperture endpoint.
 if phase==finish+1
  captured(k)=current(k);
  % Low-side OFF has no phase-current observation. Zero is an explicit
  % teaching approximation, not a calibrated amplifier switching transient.
  if cfg(2)>0 && valid(k)==0,captured(k)=0;end
  if valid(k)>0,last_good(k)=captured(k);end
  if cfg(2)>0 && cfg(3)>0 && valid(k)==0,captured(k)=last_good(k);end
 end
end
jeos=tr+3*rank;
if phase==jeos
 delivered=captured;raw_codes=min(4095,max(0,round(2048+captured/(165/4096))));pulse(5)=1;
end
sample=delivered;codes=raw_codes;
% Phase, trigger, C/B/A hold pulses, JEOS, validity ABC, sampled ABC, sum.
diag=[phase*h pulse(1:4) pulse(5) valid delivered sum(delivered) ...
       double(mod(floor(tick/N),cfg(11))==cfg(11)-1 && phase==jeos) double(phase==jeos)];
end

== matlab function PMSM_FOC_R2026a/无感观测/有效判断/瞬时相位许可 ==
  settings: updateMethod=DISCRETE  sampleTime=timing_control_sample
  data: theta input double size=1; packet_valid output boolean size=1; vector input double size=[2 1]; quality input boolean size=1; sample_valid input boolean size=1; reset input boolean size=1; cfg input double size=[1 18]; diagnostic output double size=[8 1]
function [packet_valid,diagnostic]=sless_r2_phase_guard_block(theta,vector,quality,sample_valid,reset,cfg)
%#codegen
[packet_valid,diagnostic]=sensorless_r2_phase_guard(theta,vector,quality,sample_valid,reset,cfg(16));
end
